simulink model "battery_1rc_generated"  (R2026a)
settings: Solver=FixedStepDiscrete  FixedStep=1
settings Model: Creator=savbc  LastModifiedBy=savbc

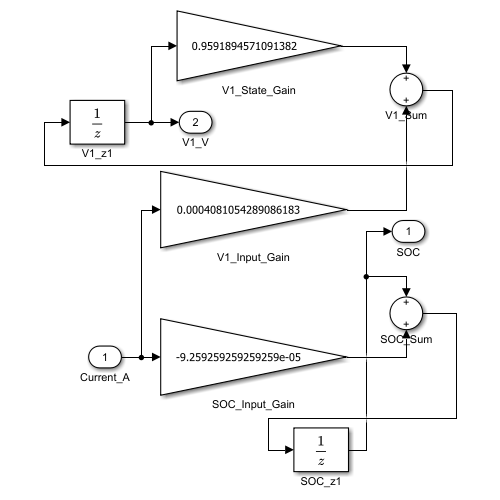
[thumbnail: Simulink's stored preview of the top-level diagram]
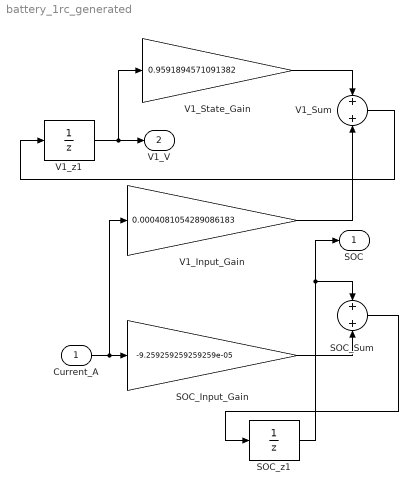
== system battery_1rc_generated ==
  Current_A : Inport
  SOC_Input_Gain : Gain  Gain=-9.259259259259259e-05
  SOC_Sum : Sum
  SOC_z1 : UnitDelay  InitialCondition=0.85
  V1_Input_Gain : Gain  Gain=0.0004081054289086183
  V1_State_Gain : Gain  Gain=0.9591894571091382
  V1_Sum : Sum
  V1_z1 : UnitDelay
  SOC : Outport
  V1_V : Outport  Port=2
  wires:
  V1_Sum/1 -> V1_z1/1
  V1_Input_Gain/1 -> V1_Sum/2
  V1_State_Gain/1 -> V1_Sum/1
  Current_A/1 -> SOC_Input_Gain/1, V1_Input_Gain/1
  V1_z1/1 -> V1_V/1, V1_State_Gain/1
  SOC_Input_Gain/1 -> SOC_Sum/2
  SOC_Sum/1 -> SOC_z1/1
  SOC_z1/1 -> SOC_Sum/1, SOC/1
